simulink model "surrogate_frictional_lag_Fvsv"  (R2026a)
settings: Solver=ode23tb  StopTime=30  MaxStep=1e-4  RelTol=1e-7  AbsTol=1e-10
undefined symbols (not defined in the file): w
settings Model: NumberOfSteps=10  Creator=kikuchi  LastModifiedBy=shuki

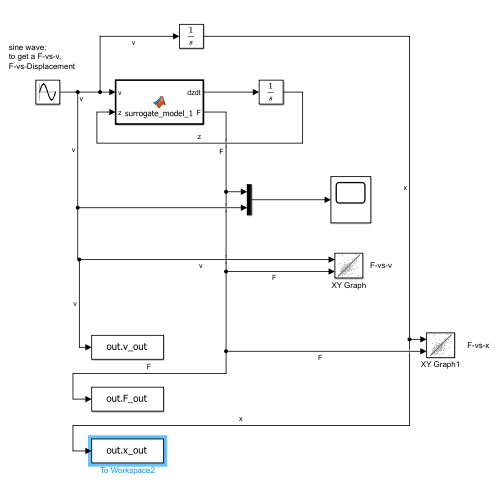
[thumbnail: Simulink's stored preview of the top-level diagram]
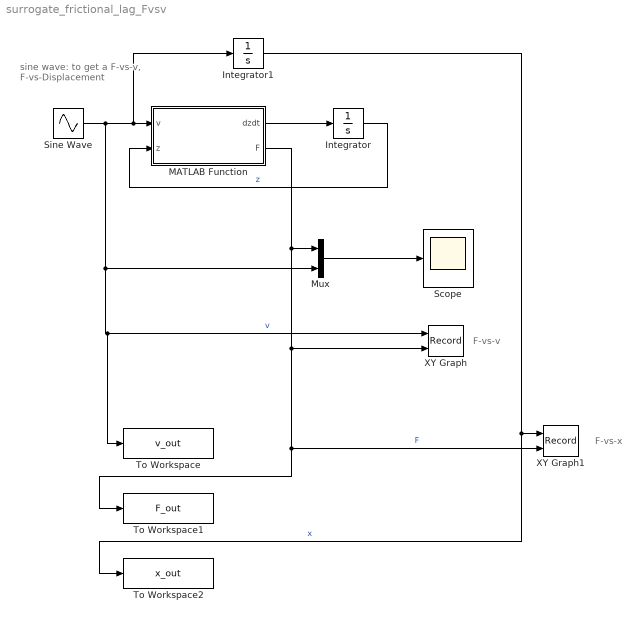
== system surrogate_frictional_lag_Fvsv ==
  note: sine wave:
      | to get a F-vs-v,
      | F-vs-Displacement
  note: F-vs-v
  note: F-vs-x
  Integrator : Integrator
  Integrator1 : Integrator
  MATLAB Function : MATLAB Function  TreatAsAtomicUnit=on
  Mux : Mux  Inputs=2
  Scope : Scope
      settings: ActiveDisplayYMinimum=-7.5445326454646242  ActiveDisplayYMaximum=4.8434715839579514
  Sine Wave : Sin  Amplitude=1e-3  Bias=1.5e-3  Frequency=w  SampleTime=0
  To Workspace : ToWorkspace  VariableName=v_out  SaveFormat=Timeseries  SampleTime=-1
  To Workspace1 : ToWorkspace  VariableName=F_out  SaveFormat=Timeseries  SampleTime=-1
  To Workspace2 : ToWorkspace  VariableName=x_out  SaveFormat=Timeseries  SampleTime=-1
  XY Graph : Record  NumPorts=2.0  FileSettingsInternal="{\"entries\":[{\"content\":{\"excelSettings\":{\"content\":{},\"type\":\"Streamout.ExcelSettings\"},\"parquetSettings\":{\"content\":{},\"type\":\"Streamout.ParquetSettings\"}},\"type\":\"Streamout.FileSettingStorage\",\"uuid\":\"\"}],\"packageUris\":[\"http:\\/\\/schema.mathworks.com\\/mf0\\/streamout_blocks\\/R2020a\"],\"version\":\"1.0\"}"  FrameSettings=[0, 0]  Layout=[1 1]  SignalsInternal="{\"entries\":[{\"content\":{\"signals\":[{\"content\":{\"blockPath\":[],\"dimensions\":[1],\"domain\":\"\",\"lineColor\":\"#a2142f\",\"plots\":[ 1 ],\"port\":1,\"sid\":[\"\"],\"signalID\":1,\"signalName\":\"v\"},\"type\":\"RecordBlkView.Signal\",\"uuid\":\"\"},{\"content\":{\"blockPath\":[],\"dimensions\":[1],\"domain\":\"\",\"lineColor\":\"#139fff\",\"plots\":[ 1 ],\"port\":2,\"sid\":[\"\"],\"signalID\":2,\"signalName\":\"F\"},\"type\":\"RecordBlkView.Signal\",\"uuid\":\"\"}]},\"type\":\"RecordBlkView.InputSignals\",\"uuid\":\"\"}],\"packageUris\":[\"http:\\/\\/schema.mathworks.com\\/mf0\\/streamout_blocks\\/R2020a\"],\"version\":\"1.0\"}"  VisualizationBindings="{\"xyplotplugin\":{\"info\":[{\"series\":[{\"bindingParametersList\":[{\"parameter\":\"X-Axis\",\"signalID\":1,\"signalName\":\"v\"},{\"parameter\":\"Y-Axis\",\"signalID\":2,\"signalName\":\"F\"}],\"seriesID\":0}],\"subplotID\":1}]}}"  CompatibilityTag=XY
  XY Graph1 : Record  NumPorts=2.0  FileSettingsInternal="{\"entries\":[{\"content\":{\"excelSettings\":{\"content\":{},\"type\":\"Streamout.ExcelSettings\"},\"parquetSettings\":{\"content\":{},\"type\":\"Streamout.ParquetSettings\"}},\"type\":\"Streamout.FileSettingStorage\",\"uuid\":\"\"}],\"packageUris\":[\"http:\\/\\/schema.mathworks.com\\/mf0\\/streamout_blocks\\/R2020a\"],\"version\":\"1.0\"}"  FrameSettings=[0, 0]  Layout=[1 1]  SignalsInternal="{\"entries\":[{\"content\":{\"signals\":[{\"content\":{\"blockPath\":[],\"dimensions\":[1],\"domain\":\"\",\"lineColor\":\"#a2142f\",\"plots\":[ 1 ],\"port\":1,\"sid\":[\"\"],\"signalID\":1,\"signalName\":\"x\"},\"type\":\"RecordBlkView.Signal\",\"uuid\":\"\"},{\"content\":{\"blockPath\":[],\"dimensions\":[1],\"domain\":\"\",\"lineColor\":\"#139fff\",\"plots\":[ 1 ],\"port\":2,\"sid\":[\"\"],\"signalID\":2,\"signalName\":\"F\"},\"type\":\"RecordBlkView.Signal\",\"uuid\":\"\"}]},\"type\":\"RecordBlkView.InputSignals\",\"uuid\":\"\"}],\"packageUris\":[\"http:\\/\\/schema.mathworks.com\\/mf0\\/streamout_blocks\\/R2020a\"],\"version\":\"1.0\"}"  VisualizationBindings="{\"xyplotplugin\":{\"info\":[{\"series\":[{\"bindingParametersList\":[{\"parameter\":\"X-Axis\",\"signalID\":1,\"signalName\":\"x\"},{\"parameter\":\"Y-Axis\",\"signalID\":2,\"signalName\":\"F\"}],\"seriesID\":0}],\"subplotID\":1}]}}"  CompatibilityTag=XY
  wires:
  Sine Wave/1 -> Integrator1/1, MATLAB Function/1(v), To Workspace/1, XY Graph/1, Mux/2  "v"
  MATLAB Function/1(dzdt) -> Integrator/1
  Integrator/1 -> MATLAB Function/2(z)  "z"
  MATLAB Function/2(F) -> XY Graph1/2, To Workspace1/1, XY Graph/2, Mux/1  "F"
  Mux/1 -> Scope/1
  Integrator1/1 -> To Workspace2/1, XY Graph1/1  "x"

== matlab function surrogate_frictional_lag_Fvsv/MATLAB Function ==
  data: v input; dzdt output; z input; F output
function [dzdt, F] = surrogate_model_16(v, z)

    S0 = 10^5;
    C1 = 32.762203;
    C2 = 55.41855;

    dzdt = v - ( abs(S0*C1*v) + (S0*v)^2 )*( z / (abs(S0*v) + C2) );

    F = 10^5 * z + 316.2277 * dzdt + 0.4 * v;

end
